simulink model "Sistema"  (R2020b)
settings: Solver=ode15s  StartTime=0.0  StopTime=10  MaxStep=1E-3  RelTol=1e-3
libraries: fl_lib x8, ee_lib x8, nesl_utility x6, pid_lib x1
settings Model: Creator=cdhan  LastModifiedBy=hiram
settings DataIOCC: SaveOutput=off  SignalLogging=off  DSMLogging=off  ReturnWorkspaceOutputs=off  TimeSaveName=t
settings DebuggingCC: AlgebraicLoopMsg=none  ArtificialAlgebraicLoopMsg=none  MaxConsecutiveZCsMsg=none  UnconnectedInputMsg=none  UnconnectedOutputMsg=none  UnconnectedLineMsg=none  ModelReferenceExtraNoncontSigs=none  OperatingPointInterfaceChecksumMismatchMsg=none
settings ModelReferenceCC: EnableRefExpFcnMdlSchedulingChecks=off

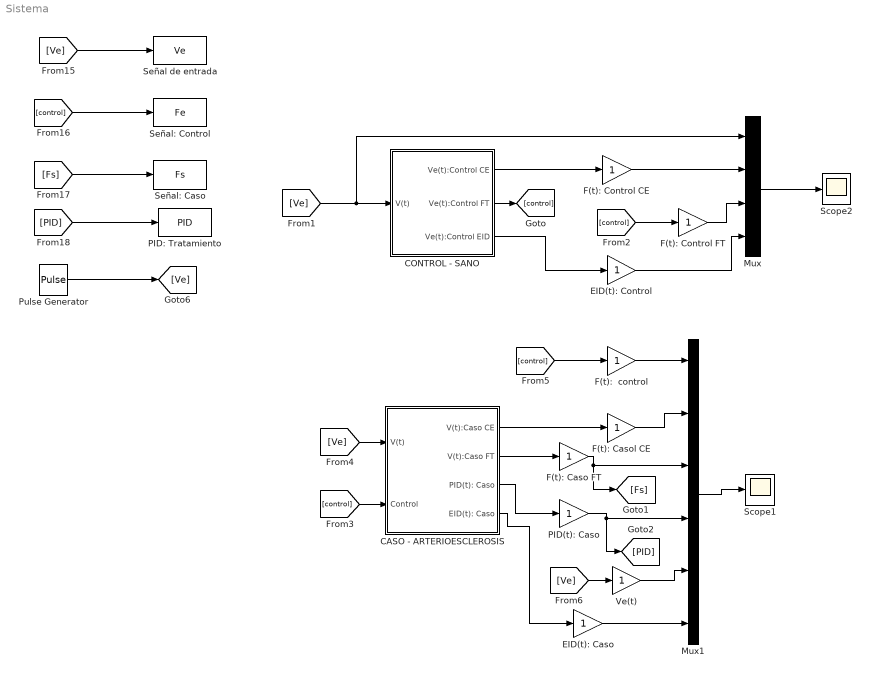
== system Sistema ==
  CASO - ARTERIOESCLEROSIS : Subsystem
  CONTROL - SANO : Subsystem
  "EID(t): Caso " : Gain
  EID(t): Control : Gain
  F(t):  control : Gain
  F(t): Caso FT : Gain
  F(t): Casol CE : Gain
  F(t): Control CE : Gain
  F(t): Control FT : Gain
  Mux : Mux
  Mux1 : Mux  Inputs=6
  "PID(t): Caso " : Gain
  PID: Tratamiento : ToWorkspace  VariableName=PID  SampleTime=-1
  Pulse Generator : DiscretePulseGenerator  PulseType=Time based  Period=10  PulseWidth=10  PhaseDelay=1
  Scope1 : Scope
  Scope2 : Scope
  Señal de entrada : ToWorkspace  VariableName=Ve  SampleTime=-1
  Señal: Caso : ToWorkspace  VariableName=Fs  SampleTime=-1
  Señal: Control : ToWorkspace  VariableName=Fe  SampleTime=-1
  "Ve(t) " : Gain
  wires:
  Mux/1 -> Scope2/1
  [control] -> Señal: Control/1
  [Fs] -> Señal: Caso/1
  Pulse Generator/1 -> [Ve]
  [Ve] -> Señal de entrada/1
  [PID] -> PID: Tratamiento/1
  [Ve] -> Mux/1, CONTROL - SANO/1(V(t))
  CONTROL - SANO/2(Ve(t):Control FT) -> [control]
  [control] -> F(t): Control FT/1
  CONTROL - SANO/1("Ve(t):Control CE ") -> F(t): Control CE/1
  [control] -> CASO - ARTERIOESCLEROSIS/2(Control)
  [Ve] -> CASO - ARTERIOESCLEROSIS/1(V(t))
  [control] -> F(t):  control/1
  CASO - ARTERIOESCLEROSIS/1(V(t):Caso CE) -> F(t): Casol CE/1
  F(t): Casol CE/1 -> Mux1/2
  CASO - ARTERIOESCLEROSIS/2(V(t):Caso FT) -> F(t): Caso FT/1
  F(t): Caso FT/1 -> [Fs], Mux1/3
  CASO - ARTERIOESCLEROSIS/3(PID(t): Caso) -> "PID(t): Caso "/1
  "PID(t): Caso "/1 -> [PID], Mux1/4
  Mux1/1 -> Scope1/1
  F(t): Control FT/1 -> Mux/3
  F(t): Control CE/1 -> Mux/2
  [Ve] -> "Ve(t) "/1
  CONTROL - SANO/3(Ve(t):Control EID) -> EID(t): Control/1
  CASO - ARTERIOESCLEROSIS/4(EID(t): Caso) -> "EID(t): Caso "/1
  "EID(t): Caso "/1 -> Mux1/6
  EID(t): Control/1 -> Mux/4
  F(t):  control/1 -> Mux1/1
  "Ve(t) "/1 -> Mux1/5

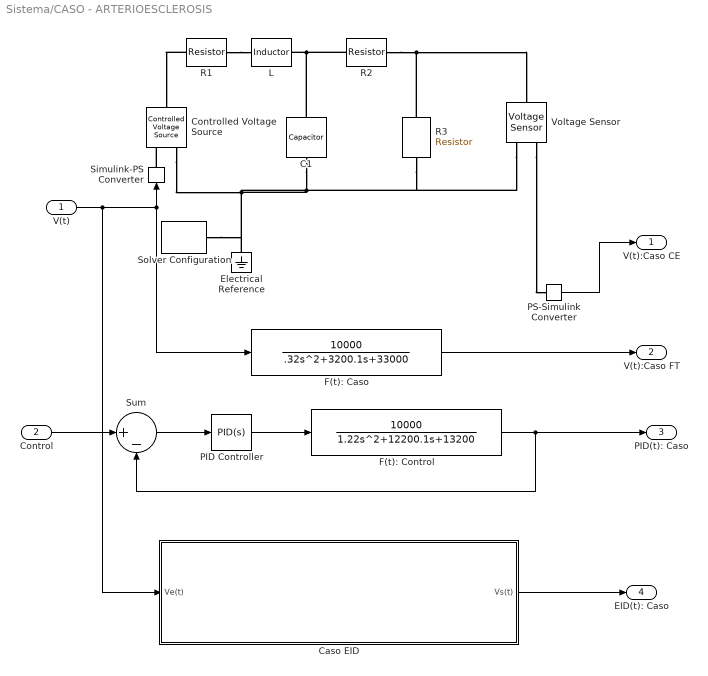
== system Sistema/CASO - ARTERIOESCLEROSIS ==
  V(t) : Inport
  Control : Inport  Port=2
  C1 : fl_lib/Electrical/Electrical Elements/Capacitor  c=100 uF  r=1e-6 Ohm  g=0 1/Ohm  i_specify=off  i_priority=None  i=0 A  i_nominal_specify=off  i_nominal_unit=A  i_nominal_value=1  v_specify=off  v_priority=None  v=0 V  v_nominal_specify=off  v_nominal_unit=V  v_nominal_value=1  vc_specify=off  vc_priority=High  vc=0 V  vc_nominal_specify=off  vc_nominal_unit=V  vc_nominal_value=1
  Caso EID : Subsystem
  Controlled Voltage Source : fl_lib/Electrical/Electrical Sources/Controlled Voltage Source
  Electrical Reference : fl_lib/Electrical/Electrical Elements/Electrical Reference
  F(t): Caso : TransferFcn  Numerator=10000  Denominator=[.32, 3200.1,33000]
  F(t): Control : TransferFcn  Numerator=10000  Denominator=[1.22, 12200.1,13200]
  L : ee_lib/Passive/Inductor  l=100 mH  L_tol=20  enable_L_tol=0  tol_distribution=1  nSigma=4  r=0 Ohm  g=1e-9 1/Ohm  enable_operating_limits=0  operating_limit_action=2  max_working_current=1 A  power_rating=1 W  enable_faults=0  fault_action=1  lambdaPercent=50  k_faulted=0.9999  turnsShort=0  openCct=0  groundShort=0  groundShortG=0 1/Ohm  tau_fault=1e-3 s  enable_temporal_fault=0  t_fault=1 s  enable_behavioral_fault=0  max_permissible_voltage=100 V  n_fail_on_voltage=1  max_permissible_current=1 A  t_fail_on_current=1 s  i_L_specify=off  i_L_priority=High  i_L=0 A  i_L_nominal_specify=off  i_L_nominal_unit=A  i_L_nominal_value=1
  PID Controller : pid_lib/PID Controller  Controller=PID  Form=Parallel  TimeDomain=Continuous-time  UseExternalTs=off  SampleTime=-1  IntegratorMethod=Forward Euler  FilterMethod=Forward Euler  ControllerParametersSource=internal  P=26370.7413010644  I=43149447.1245296  D=2.77989475348095  UseFilter=on  N=2520772.12224817  TunerSelectOption=Transfer Function Based (PID Tuner App)  InitialConditionSource=internal  InitialConditionForIntegrator=0  InitialConditionForFilter=0  DifferentiatorICPrevScaledInput=0  ExternalReset=none  TrackingMode=off  Kt=1  LimitOutput=off  SatLimitsSource=internal  UpperSaturationLimit=inf  LowerSaturationLimit=-inf  LinearizeAsGain=on  AntiWindupMode=none  Kb=1  POutMin=[]  POutMax=[]  IOutMin=[]  IOutMax=[]  DOutMin=[]  DOutMax=[]  NOutMin=[]  NOutMax=[]  SumOutMin=[]  SumOutMax=[]  SaturationOutMin=[]  SaturationOutMax=[]  PParamMin=[]  PParamMax=[]  IParamMin=[]  IParamMax=[]  DParamMin=[]  DParamMax=[]  NParamMin=[]  NParamMax=[]  KbParamMin=[]  KbParamMax=[]  KtParamMin=[]  KtParamMax=[]  KbOutMin=[]  KbOutMax=[]  KtOutMin=[]  KtOutMax=[]  IntegratorOutMin=[]  IntegratorOutMax=[]  FilterOutMin=[]  FilterOutMax=[]  SumI1OutMin=[]  SumI1OutMax=[]  SumI2OutMin=[]  SumI2OutMax=[]  SumI3OutMin=[]  SumI3OutMax=[]  SumI4OutMin=[]  SumI4OutMax=[]  SumDOutMin=[]  SumDOutMax=[]  DifferentiatorOutMin=[]  DifferentiatorOutMax=[]  FilterDiffOutCoefMin=[]  FilterDiffOutCoefMax=[]  ReciprocalOutMin=[]  ReciprocalOutMax=[]  SumDenOutMin=[]  SumDenOutMax=[]  SumNumOutMin=[]  SumNumOutMax=[]  DivideOutMin=[]  DivideOutMax=[]  UdiffTsProdOutMin=[]  UdiffTsProdOutMax=[]  NTsProdOutMin=[]  NTsProdOutMax=[]  UintegralTsProdOutMin=[]  UintegralTsProdOutMax=[]  UngainTsProdOutMin=[]  UngainTsProdOutMax=[]  IntegratorContinuousStateAttributes=''  IntegratorStateMustResolveToSignalObject=off  IntegratorRTWStateStorageClass=Auto  FilterContinuousStateAttributes=''  FilterStateMustResolveToSignalObject=off  FilterRTWStateStorageClass=Auto  ParallelPVariant=InternalParameters  IdealPVariant=Disabled  IVariant=InternalParameters  DVariant=InternalParameters  IntegratorVariant=Continuous  SatVariant=Disabled  AWVariant=Passthrough  PCopyVariant=Disabled  TRVariant=Disabled  FdbkBlocksVariant=Forward  IdealPFdbkVariant=Disabled  SatFdbkVariant=Disabled  DerivativeFilterVariant=ContFilter  NVariant=InternalParameters  NCopyVariant=Disabled  FilterICVariant=InternalICsFilter  IntegratorICVariant=InternalICs  ExternalResetVariant=Disabled  TRSumVariant=Passthrough  SumFdbkVariant=Disabled  SumVariant=Sum_PID  TsampFilterVariant=InternalTs  TsampNgainVariant=Passthrough  TsampIntegralVariant=Passthrough  ExternalSaturationOutDataTypeStr=Inherit: Same as second input
  PS-Simulink Converter : nesl_utility/PS-Simulink Converter  PhysicalDomain=network_engine_domain  SubClassName=ps_output  LeftPortType=input  RightPortType=output  PseudoPeriodic=off  Frequencies=[]  Unit=inherit  AffineConversion=off
  R1 : ee_lib/Passive/Resistor  R=1 kOhm  R_tol=5  enable_R_tol=0  tol_distribution=1  nSigma=4  enable_operating_limits=0  operating_limit_action=2  max_working_voltage=100 V  power_rating=1 W  enable_faults=0  fault_action=1  R_faulted=inf Ohm  enable_temporal_fault=0  t_fault=1 s  enable_behavioral_fault=0  max_permissible_current=1 A  t_fail_on_current=1 s  noise_mode=0  sample_time=1e-3 s  repeatability=1  auto_seed=2353087603  user_seed=0  Tdevice=25 degC  alpha=3.93e-3 1/K  Tmeas=25 degC  thermal_mass=100 J/K  power_derating_T1=70 degC  power_derating_T2=155 degC  operating_temperature_range_vec=[-50, 150] degC  temperature_specify=off  temperature_priority=High  temperature=298.15 K  temperature_nominal_specify=off  temperature_nominal_unit=K  temperature_nominal_value=1
  R2 : ee_lib/Passive/Resistor  R=22 kOhm  R_tol=5  enable_R_tol=0  tol_distribution=1  nSigma=4  enable_operating_limits=0  operating_limit_action=2  max_working_voltage=100 V  power_rating=1 W  enable_faults=0  fault_action=1  R_faulted=inf Ohm  enable_temporal_fault=0  t_fault=1 s  enable_behavioral_fault=0  max_permissible_current=1 A  t_fail_on_current=1 s  noise_mode=0  sample_time=1e-3 s  repeatability=1  auto_seed=4049024516  user_seed=0  Tdevice=25 degC  alpha=3.93e-3 1/K  Tmeas=25 degC  thermal_mass=100 J/K  power_derating_T1=70 degC  power_derating_T2=155 degC  operating_temperature_range_vec=[-50, 150] degC  temperature_specify=off  temperature_priority=High  temperature=298.15 K  temperature_nominal_specify=off  temperature_nominal_unit=K  temperature_nominal_value=1
  R3 : ee_lib/Passive/Resistor  R=10 kOhm  R_tol=5  enable_R_tol=0  tol_distribution=1  nSigma=4  enable_operating_limits=0  operating_limit_action=2  max_working_voltage=100 V  power_rating=1 W  enable_faults=0  fault_action=1  R_faulted=inf Ohm  enable_temporal_fault=0  t_fault=1 s  enable_behavioral_fault=0  max_permissible_current=1 A  t_fail_on_current=1 s  noise_mode=0  sample_time=1e-3 s  repeatability=1  auto_seed=2293787961  user_seed=0  Tdevice=25 degC  alpha=3.93e-3 1/K  Tmeas=25 degC  thermal_mass=100 J/K  power_derating_T1=70 degC  power_derating_T2=155 degC  operating_temperature_range_vec=[-50, 150] degC  temperature_specify=off  temperature_priority=High  temperature=298.15 K  temperature_nominal_specify=off  temperature_nominal_unit=K  temperature_nominal_value=1
  Simulink-PS Converter : nesl_utility/Simulink-PS Converter  PhysicalDomain=network_engine_domain  SubClassName=ps_input  LeftPortType=input  RightPortType=output  PseudoPeriodic=off  Frequencies=[]  NoiseDistribution=none  NoiseParameters=[]  Unit=1  AffineConversion=off  FilteringAndDerivatives=provide  SimscapeFilterOrder=1  InputFilterTimeConstant=0.001  UdotUserProvided=0
  Solver Configuration : nesl_utility/Solver Configuration  PhysicalDomain=network_engine_domain  SubClassName=solver  LeftPortType=input  RightPortType=generic  Tones=[]  Harmonics=[]  SimulateNoise=off  Profile=off  UseLocalSampling=off  EnableSwitchedLinearOptims=on  FrequencyDomain=off  UseCCode=off  RelTol=0.001  AbsTol=1e-06  MinStep=1e-09  ToWorkspace=off  RevertToSquareIcSolve=off  NumHomotopyIterations=100  PhasorMode=off  PhasorModeNumHarmonics=1  DoDC=off  ResidualTolerance=1e-09  UseLocalSolver=off  LocalSolverChoice=NE_BACKWARD_EULER_ADVANCER  LocalSolverSampleTime=0.001  DoFixedCost=off  MaxNonlinIter=3  MaxModeIter=2  ComputeImpulses=off  ImpulseIterations=2  LinearAlgebra=auto  EquationFormulation=NE_TIME_EF  DelaysMemoryBudget=1024  AutomaticFiltering=on  FilteringTimeConstant=0.001  PartitionStorageMethod=AS_NEEDED  PartitionMemoryBudget=1024  PartitionMethod=ROBUST
  Sum : Sum  Inputs=|+-
  Voltage Sensor : fl_lib/Electrical/Electrical Sensors/Voltage Sensor
  V(t):Caso CE : Outport
  V(t):Caso FT : Outport  Port=2
  PID(t): Caso : Outport  Port=3
  EID(t): Caso : Outport  Port=4
  wires:
  PS-Simulink Converter/1 -> V(t):Caso CE/1
  V(t)/1 -> Caso EID/1(Ve(t)), Simulink-PS Converter/1, F(t): Caso/1
  F(t): Caso/1 -> V(t):Caso FT/1
  PID Controller/1 -> F(t): Control/1
  Control/1 -> Sum/1
  F(t): Control/1 -> Sum/2, PID(t): Caso/1
  Sum/1 -> PID Controller/1
  Caso EID/1(Vs(t)) -> EID(t): Caso/1
  connections:
  R2/RConn1 -- R3/LConn1 -- Voltage Sensor/LConn1
  Controlled Voltage Source/RConn2 -- Electrical Reference/LConn1 -- Solver Configuration/RConn1 -- R3/RConn1 -- Voltage Sensor/RConn2 -- C1/RConn1
  R1/LConn1 -- Controlled Voltage Source/LConn1
  Voltage Sensor/RConn1 -- PS-Simulink Converter/LConn1
  Simulink-PS Converter/RConn1 -- Controlled Voltage Source/RConn1
  C1/LConn1 -- R2/LConn1 -- L/RConn1
  R1/RConn1 -- L/LConn1

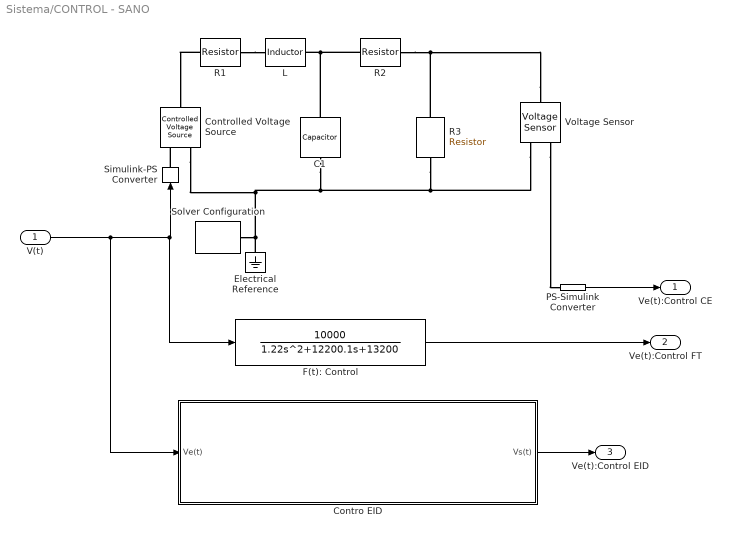
== system Sistema/CONTROL - SANO ==
  V(t) : Inport
  C1 : fl_lib/Electrical/Electrical Elements/Capacitor  c=1000 uF  r=1e-6 Ohm  g=0 1/Ohm  i_specify=off  i_priority=None  i=0 A  i_nominal_specify=off  i_nominal_unit=A  i_nominal_value=1  v_specify=off  v_priority=None  v=0 V  v_nominal_specify=off  v_nominal_unit=V  v_nominal_value=1  vc_specify=off  vc_priority=High  vc=0 V  vc_nominal_specify=off  vc_nominal_unit=V  vc_nominal_value=1
  Contro EID : Subsystem
  Controlled Voltage Source : fl_lib/Electrical/Electrical Sources/Controlled Voltage Source
  Electrical Reference : fl_lib/Electrical/Electrical Elements/Electrical Reference
  F(t): Control : TransferFcn  Numerator=10000  Denominator=[1.22, 12200.1,13200]
  L : ee_lib/Passive/Inductor  l=100 mH  L_tol=20  enable_L_tol=0  tol_distribution=1  nSigma=4  r=0 Ohm  g=1e-9 1/Ohm  enable_operating_limits=0  operating_limit_action=2  max_working_current=1 A  power_rating=1 W  enable_faults=0  fault_action=1  lambdaPercent=50  k_faulted=0.9999  turnsShort=0  openCct=0  groundShort=0  groundShortG=0 1/Ohm  tau_fault=1e-3 s  enable_temporal_fault=0  t_fault=1 s  enable_behavioral_fault=0  max_permissible_voltage=100 V  n_fail_on_voltage=1  max_permissible_current=1 A  t_fail_on_current=1 s  i_L_specify=off  i_L_priority=High  i_L=0 A  i_L_nominal_specify=off  i_L_nominal_unit=A  i_L_nominal_value=1
  PS-Simulink Converter : nesl_utility/PS-Simulink Converter  PhysicalDomain=network_engine_domain  SubClassName=ps_output  LeftPortType=input  RightPortType=output  PseudoPeriodic=off  Frequencies=[]  Unit=inherit  AffineConversion=off
  R1 : ee_lib/Passive/Resistor  R=1 kOhm  R_tol=5  enable_R_tol=0  tol_distribution=1  nSigma=4  enable_operating_limits=0  operating_limit_action=2  max_working_voltage=100 V  power_rating=1 W  enable_faults=0  fault_action=1  R_faulted=inf Ohm  enable_temporal_fault=0  t_fault=1 s  enable_behavioral_fault=0  max_permissible_current=1 A  t_fail_on_current=1 s  noise_mode=0  sample_time=1e-3 s  repeatability=1  auto_seed=386335224  user_seed=0  Tdevice=25 degC  alpha=3.93e-3 1/K  Tmeas=25 degC  thermal_mass=100 J/K  power_derating_T1=70 degC  power_derating_T2=155 degC  operating_temperature_range_vec=[-50, 150] degC  temperature_specify=off  temperature_priority=High  temperature=298.15 K  temperature_nominal_specify=off  temperature_nominal_unit=K  temperature_nominal_value=1
  R2 : ee_lib/Passive/Resistor  R=2.2 kOhm  R_tol=5  enable_R_tol=0  tol_distribution=1  nSigma=4  enable_operating_limits=0  operating_limit_action=2  max_working_voltage=100 V  power_rating=1 W  enable_faults=0  fault_action=1  R_faulted=inf Ohm  enable_temporal_fault=0  t_fault=1 s  enable_behavioral_fault=0  max_permissible_current=1 A  t_fail_on_current=1 s  noise_mode=0  sample_time=1e-3 s  repeatability=1  auto_seed=479772518  user_seed=0  Tdevice=25 degC  alpha=3.93e-3 1/K  Tmeas=25 degC  thermal_mass=100 J/K  power_derating_T1=70 degC  power_derating_T2=155 degC  operating_temperature_range_vec=[-50, 150] degC  temperature_specify=off  temperature_priority=High  temperature=298.15 K  temperature_nominal_specify=off  temperature_nominal_unit=K  temperature_nominal_value=1
  R3 : ee_lib/Passive/Resistor  R=10 kOhm  R_tol=5  enable_R_tol=0  tol_distribution=1  nSigma=4  enable_operating_limits=0  operating_limit_action=2  max_working_voltage=100 V  power_rating=1 W  enable_faults=0  fault_action=1  R_faulted=inf Ohm  enable_temporal_fault=0  t_fault=1 s  enable_behavioral_fault=0  max_permissible_current=1 A  t_fail_on_current=1 s  noise_mode=0  sample_time=1e-3 s  repeatability=1  auto_seed=585372041  user_seed=0  Tdevice=25 degC  alpha=3.93e-3 1/K  Tmeas=25 degC  thermal_mass=100 J/K  power_derating_T1=70 degC  power_derating_T2=155 degC  operating_temperature_range_vec=[-50, 150] degC  temperature_specify=off  temperature_priority=High  temperature=298.15 K  temperature_nominal_specify=off  temperature_nominal_unit=K  temperature_nominal_value=1
  Simulink-PS Converter : nesl_utility/Simulink-PS Converter  PhysicalDomain=network_engine_domain  SubClassName=ps_input  LeftPortType=input  RightPortType=output  PseudoPeriodic=off  Frequencies=[]  NoiseDistribution=none  NoiseParameters=[]  Unit=1  AffineConversion=off  FilteringAndDerivatives=provide  SimscapeFilterOrder=1  InputFilterTimeConstant=0.001  UdotUserProvided=0
  Solver Configuration : nesl_utility/Solver Configuration  PhysicalDomain=network_engine_domain  SubClassName=solver  LeftPortType=input  RightPortType=generic  Tones=[]  Harmonics=[]  SimulateNoise=off  Profile=off  UseLocalSampling=off  EnableSwitchedLinearOptims=on  FrequencyDomain=off  UseCCode=off  RelTol=0.001  AbsTol=1e-06  MinStep=1e-09  ToWorkspace=off  RevertToSquareIcSolve=off  NumHomotopyIterations=100  PhasorMode=off  PhasorModeNumHarmonics=1  DoDC=off  ResidualTolerance=1e-09  UseLocalSolver=off  LocalSolverChoice=NE_BACKWARD_EULER_ADVANCER  LocalSolverSampleTime=0.001  DoFixedCost=off  MaxNonlinIter=3  MaxModeIter=2  ComputeImpulses=off  ImpulseIterations=2  LinearAlgebra=auto  EquationFormulation=NE_TIME_EF  DelaysMemoryBudget=1024  AutomaticFiltering=on  FilteringTimeConstant=0.001  PartitionStorageMethod=AS_NEEDED  PartitionMemoryBudget=1024  PartitionMethod=ROBUST
  Voltage Sensor : fl_lib/Electrical/Electrical Sensors/Voltage Sensor
  "Ve(t):Control CE " : Outport
  Ve(t):Control FT : Outport  Port=2
  Ve(t):Control EID : Outport  Port=3
  wires:
  F(t): Control/1 -> Ve(t):Control FT/1
  PS-Simulink Converter/1 -> "Ve(t):Control CE "/1
  Contro EID/1(Vs(t)) -> Ve(t):Control EID/1
  V(t)/1 -> Contro EID/1(Ve(t)), F(t): Control/1, Simulink-PS Converter/1
  connections:
  L/RConn1 -- C1/LConn1 -- R2/LConn1
  Solver Configuration/RConn1 -- Controlled Voltage Source/RConn2 -- R3/RConn1 -- Voltage Sensor/RConn2 -- C1/RConn1 -- Electrical Reference/LConn1
  Voltage Sensor/LConn1 -- R3/LConn1 -- R2/RConn1
  Simulink-PS Converter/RConn1 -- Controlled Voltage Source/RConn1
  R1/RConn1 -- L/LConn1
  R1/LConn1 -- Controlled Voltage Source/LConn1
  Voltage Sensor/RConn1 -- PS-Simulink Converter/LConn1

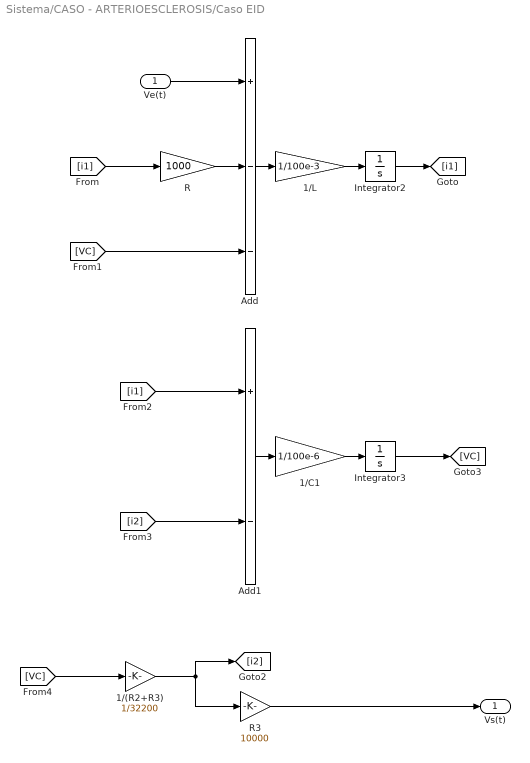
== system Sistema/CASO - ARTERIOESCLEROSIS/Caso EID ==
  Ve(t) : Inport
  1/(R2+R3) : Gain  Gain=1/32200
  1/C1 : Gain  Gain=1/100e-6
  1/L : Gain  Gain=1/100e-3
  Add : Sum  Inputs=+--
  Add1 : Sum  Inputs=+-
  Integrator2 : Integrator
  Integrator3 : Integrator
  R : Gain  Gain=1000
  R3 : Gain  Gain=10000
  Vs(t) : Outport
  wires:
  R/1 -> Add/2
  Ve(t)/1 -> Add/1
  [i1] -> R/1
  Add/1 -> 1/L/1
  1/L/1 -> Integrator2/1
  Integrator2/1 -> [i1]
  [VC] -> Add/3
  1/C1/1 -> Integrator3/1
  Add1/1 -> 1/C1/1
  Integrator3/1 -> [VC]
  [i2] -> Add1/2
  [i1] -> Add1/1
  [VC] -> 1/(R2+R3)/1
  1/(R2+R3)/1 -> R3/1, [i2]
  R3/1 -> Vs(t)/1

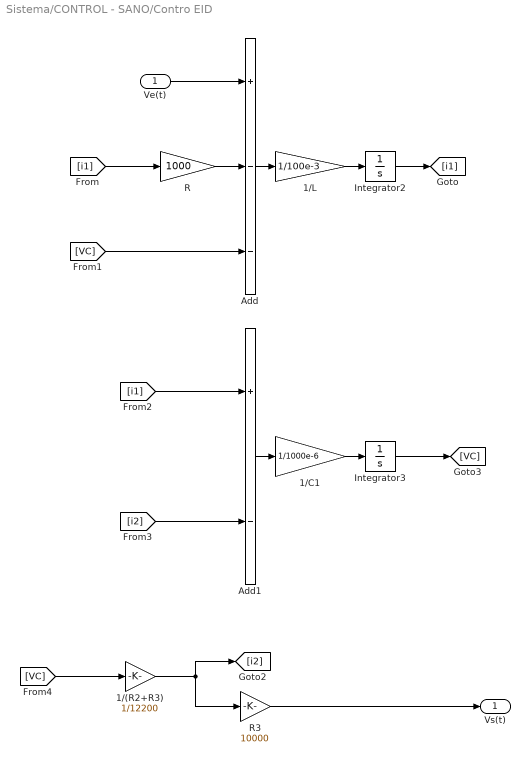
== system Sistema/CONTROL - SANO/Contro EID ==
  Ve(t) : Inport
  1/(R2+R3) : Gain  Gain=1/12200
  1/C1 : Gain  Gain=1/1000e-6
  1/L : Gain  Gain=1/100e-3
  Add : Sum  Inputs=+--
  Add1 : Sum  Inputs=+-
  Integrator2 : Integrator
  Integrator3 : Integrator
  R : Gain  Gain=1000
  R3 : Gain  Gain=10000
  Vs(t) : Outport
  wires:
  R/1 -> Add/2
  Ve(t)/1 -> Add/1
  [i1] -> R/1
  Add/1 -> 1/L/1
  1/L/1 -> Integrator2/1
  Integrator2/1 -> [i1]
  [VC] -> Add/3
  1/C1/1 -> Integrator3/1
  Add1/1 -> 1/C1/1
  Integrator3/1 -> [VC]
  [i2] -> Add1/2
  [i1] -> Add1/1
  [VC] -> 1/(R2+R3)/1
  1/(R2+R3)/1 -> R3/1, [i2]
  R3/1 -> Vs(t)/1
